simulink model "lab6_task4_model2optimized"  (R2024b)
settings: Solver=ode45  StartTime=0.0  StopTime=10.0  MaxStep=0.01  RelTol=1e-3
settings Model: Creator=Beanie  LastModifiedBy=Beanie

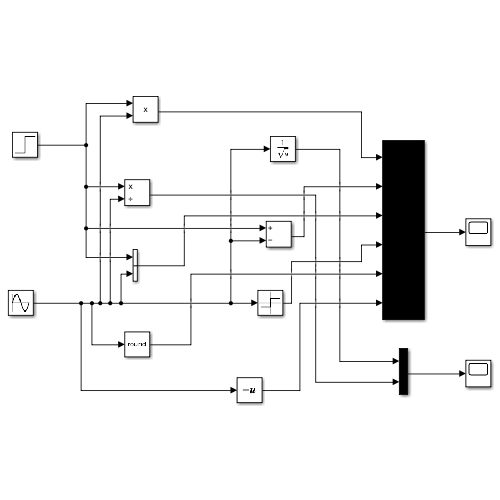
[thumbnail: Simulink's stored preview of the top-level diagram]
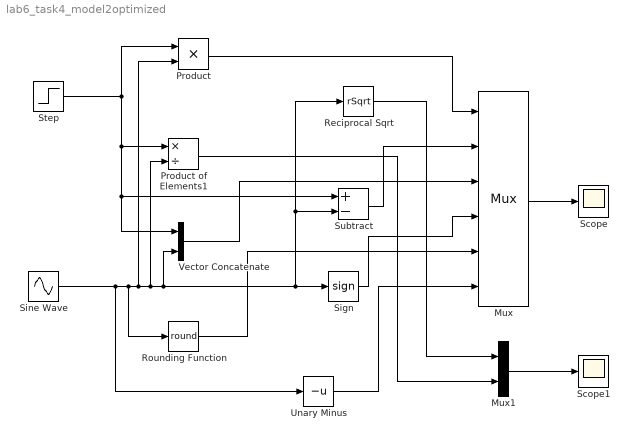
== system lab6_task4_model2optimized ==
  Mux : Mux  Inputs=6
  Mux1 : Mux  Inputs=2
  Product : Product
  Product of Elements1 : Product  Inputs=*/
  Reciprocal Sqrt : Sqrt  Operator=rSqrt
  Rounding Function : Rounding  Operator=round
  Scope : Scope
  Scope1 : Scope
  Sign : Signum
  Sine Wave : Sin  Frequency=2*pi  SampleTime=0
  Step : Step  SampleTime=0
  Subtract : Sum  Inputs=+-
  Unary Minus : UnaryMinus
  Vector Concatenate : Concatenate
  wires:
  Step/1 -> Vector Concatenate/1, Subtract/1, Product of Elements1/1, Product/1
  Sine Wave/1 -> Unary Minus/1, Rounding Function/1, Product/2, Product of Elements1/2, Vector Concatenate/2, Reciprocal Sqrt/1, Subtract/2, Sign/1
  Mux/1 -> Scope/1
  Mux1/1 -> Scope1/1
  Reciprocal Sqrt/1 -> Mux1/1
  Product of Elements1/1 -> Mux1/2
  Unary Minus/1 -> Mux/6
  Rounding Function/1 -> Mux/5
  Sign/1 -> Mux/4
  Vector Concatenate/1 -> Mux/3
  Subtract/1 -> Mux/2
  Product/1 -> Mux/1
